simulink model "elp_actuators"  (R2026b)
settings: Solver=VariableStepAuto
undefined symbols (not defined in the file or in its folder): P, Ts
libraries: simulink x1
settings Model: Creator=aomar  LastModifiedBy=aomar

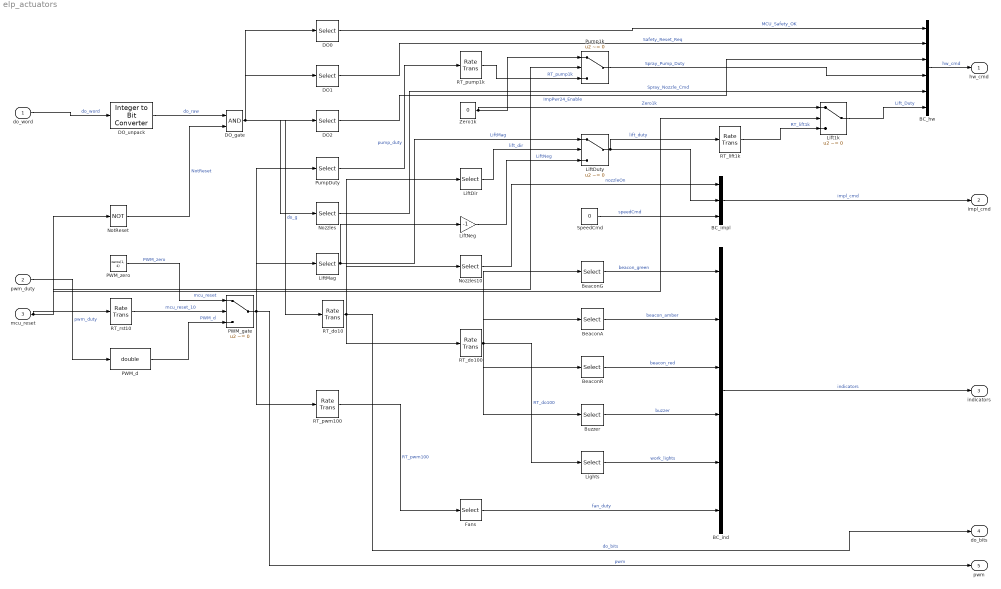
== system elp_actuators ==
  do_word : Inport  OutDataTypeStr=uint32  SampleTime=Ts.base
  pwm_duty : Inport  Port=2  OutDataTypeStr=single  PortDimensions=4  SampleTime=Ts.ctrl
  mcu_reset : Inport  Port=3  OutDataTypeStr=boolean  SampleTime=Ts.base
  BC_hw : BusCreator  Inputs=6  OutDataTypeStr=Bus: Bus_PowerHwCmd  NonVirtualBus=on
      settings: InheritFromInputs=off
  BC_impl : BusCreator  Inputs=3  OutDataTypeStr=Bus: Bus_ImplementCmd  NonVirtualBus=on
      settings: InheritFromInputs=off
  BC_ind : BusCreator  Inputs=6  OutDataTypeStr=Bus: Bus_IndicatorOut  NonVirtualBus=on
      settings: InheritFromInputs=off
  BeaconA : Selector  InputPortWidth=32  IndexOptions=Index vector (dialog)  Indices=1 + P.electronics.do.beacon_amber  OutputSizes=1
  BeaconG : Selector  InputPortWidth=32  IndexOptions=Index vector (dialog)  Indices=1 + P.electronics.do.beacon_green  OutputSizes=1
  BeaconR : Selector  InputPortWidth=32  IndexOptions=Index vector (dialog)  Indices=1 + P.electronics.do.beacon_red  OutputSizes=1
  Buzzer : Selector  InputPortWidth=32  IndexOptions=Index vector (dialog)  Indices=1 + P.electronics.do.buzzer  OutputSizes=1
  DO0 : Selector  InputPortWidth=32  IndexOptions=Index vector (dialog)  Indices=1 + P.electronics.do.mcu_safety_ok  OutputSizes=1
  DO1 : Selector  InputPortWidth=32  IndexOptions=Index vector (dialog)  Indices=1 + P.electronics.do.safety_reset_req  OutputSizes=1
  DO2 : Selector  InputPortWidth=32  IndexOptions=Index vector (dialog)  Indices=1 + P.electronics.do.impl24_en  OutputSizes=1
  DO_gate : Logic  AllPortsSameDT=off  OutDataTypeStr=boolean
  DO_unpack : simulink/Logic and Bit Operations/Integer to Bit Converter  nbits=32  signedInputValues=Unsigned  bitOrder=LSB first  outDtype=boolean
      settings: LibrarySourceBlock=|
      | commutil2/Integer to Bit
      | Converter
  Fans : Selector  InputPortWidth=4  IndexOptions=Index vector (dialog)  Indices=[3 4]  OutputSizes=1
  Lift1k : Switch  Criteria=u2 ~= 0  SaturateOnIntegerOverflow=off  InputSameDT=off
  LiftDir : Selector  InputPortWidth=32  IndexOptions=Index vector (dialog)  Indices=1 + P.electronics.do.lift_dir  OutputSizes=1
  LiftDuty : Switch  Criteria=u2 ~= 0  SaturateOnIntegerOverflow=off  InputSameDT=off
  LiftMag : Selector  InputPortWidth=4  IndexOptions=Index vector (dialog)  Indices=2  OutputSizes=1
  LiftNeg : Gain  Gain=-1
  Lights : Selector  InputPortWidth=32  IndexOptions=Index vector (dialog)  Indices=1 + P.electronics.do.work_lights  OutputSizes=1
  NotReset : Logic  Operator=NOT  Inputs=1  AllPortsSameDT=off  OutDataTypeStr=boolean
  Nozzles : Selector  InputPortWidth=32  IndexOptions=Index vector (dialog)  Indices=1 + P.electronics.do.nozzle1 + (0:7)  OutputSizes=1
  Nozzles10 : Selector  InputPortWidth=32  IndexOptions=Index vector (dialog)  Indices=1 + P.electronics.do.nozzle1 + (0:7)  OutputSizes=1
  PWM_d : DataTypeConversion  OutDataTypeStr=double  RndMeth=Nearest
  PWM_gate : Switch  Criteria=u2 ~= 0  SaturateOnIntegerOverflow=off  InputSameDT=off
  PWM_zero : Constant  Value=zeros(1, 4)  OutDataTypeStr=double  SampleTime=Ts.ctrl
  Pump1k : Switch  Criteria=u2 ~= 0  SaturateOnIntegerOverflow=off  InputSameDT=off
  PumpDuty : Selector  InputPortWidth=4  IndexOptions=Index vector (dialog)  Indices=1  OutputSizes=1
  RT_do10 : RateTransition  InitialCondition=false  OutPortSampleTime=Ts.ctrl
  RT_do100 : RateTransition  InitialCondition=false  OutPortSampleTime=Ts.hk
  RT_lift1k : RateTransition  OutPortSampleTime=Ts.base
  RT_pump1k : RateTransition  OutPortSampleTime=Ts.base
  RT_pwm100 : RateTransition  OutPortSampleTime=Ts.hk
  RT_rst10 : RateTransition  InitialCondition=false  OutPortSampleTime=Ts.ctrl
  SpeedCmd : Constant  Value=0  OutDataTypeStr=double  SampleTime=Ts.ctrl
  Zero1k : Constant  Value=0  OutDataTypeStr=double  SampleTime=Ts.base
  hw_cmd : Outport  OutDataTypeStr=Bus: Bus_PowerHwCmd
  impl_cmd : Outport  Port=2  OutDataTypeStr=Bus: Bus_ImplementCmd
  indicators : Outport  Port=3  OutDataTypeStr=Bus: Bus_IndicatorOut
  do_bits : Outport  Port=4  OutDataTypeStr=boolean
  pwm : Outport  Port=5  OutDataTypeStr=double
  wires:
  do_word/1 -> DO_unpack/1  "do_word"
  pwm_duty/1 -> PWM_d/1  "pwm_duty"
  mcu_reset/1 -> Pump1k/2, Lift1k/2, NotReset/1, RT_rst10/1  "mcu_reset"
  NotReset/1 -> DO_gate/2  "NotReset"
  PWM_zero/1 -> PWM_gate/1  "PWM_zero"
  RT_rst10/1 -> PWM_gate/2  "mcu_reset_10"
  PWM_d/1 -> PWM_gate/3  "PWM_d"
  DO_unpack/1 -> DO_gate/1  "do_raw"
  DO_gate/1 -> RT_do10/1, Nozzles/1, DO0/1, DO1/1, DO2/1  "do_g"
  PWM_gate/1 -> pwm/1, PumpDuty/1, RT_pwm100/1, LiftMag/1  "pwm"
  DO0/1 -> BC_hw/1  "MCU_Safety_OK"
  DO1/1 -> BC_hw/2  "Safety_Reset_Req"
  DO2/1 -> BC_hw/3  "ImpPwr24_Enable"
  PumpDuty/1 -> RT_pump1k/1  "pump_duty"
  Nozzles/1 -> BC_hw/5  "Spray_Nozzle_Cmd"
  LiftMag/1 -> LiftDuty/1, LiftNeg/1  "LiftMag"
  RT_pwm100/1 -> Fans/1  "RT_pwm100"
  RT_do10/1 -> do_bits/1, LiftDir/1, Nozzles10/1, RT_do100/1  "do_bits"
  Zero1k/1 -> Pump1k/1, Lift1k/1  "Zero1k"
  LiftNeg/1 -> LiftDuty/3  "LiftNeg"
  RT_pump1k/1 -> Pump1k/3  "RT_pump1k"
  LiftDir/1 -> LiftDuty/2  "lift_dir"
  Nozzles10/1 -> BC_impl/1  "nozzleOn"
  RT_do100/1 -> Lights/1, BeaconG/1, Buzzer/1, BeaconA/1, BeaconR/1  "RT_do100"
  Fans/1 -> BC_ind/6  "fan_duty"
  SpeedCmd/1 -> BC_impl/3  "speedCmd"
  BeaconG/1 -> BC_ind/1  "beacon_green"
  BeaconA/1 -> BC_ind/2  "beacon_amber"
  BeaconR/1 -> BC_ind/3  "beacon_red"
  Buzzer/1 -> BC_ind/4  "buzzer"
  Lights/1 -> BC_ind/5  "work_lights"
  Pump1k/1 -> BC_hw/4  "Spray_Pump_Duty"
  LiftDuty/1 -> BC_impl/2, RT_lift1k/1  "lift_duty"
  BC_impl/1 -> impl_cmd/1  "impl_cmd"
  BC_ind/1 -> indicators/1  "indicators"
  RT_lift1k/1 -> Lift1k/3  "RT_lift1k"
  Lift1k/1 -> BC_hw/6  "Lift_Duty"
  BC_hw/1 -> hw_cmd/1  "hw_cmd"
